simulink model "servomotor_pendul"  (Simulink 6.6)
settings: Solver=ode45  StartTime=0.0  StopTime=10  RelTol=1e-3
settings Model: Creator=123  LastModifiedBy=123

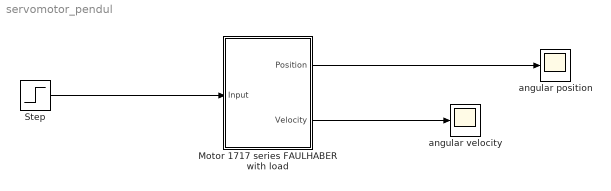
== system servomotor_pendul ==
  Motor 1717 series FAULHABER with load : Subsystem
  Step : Step  SampleTime=0
  angular position : Scope
  angular velocity : Scope
      settings: SaveName=ScopeData2
  wires:
  Step/1 -> Motor 1717 series FAULHABER with load/1(Input)
  Motor 1717 series FAULHABER with load/1(Position) -> angular position/1
  Motor 1717 series FAULHABER with load/2(Velocity) -> angular velocity/1

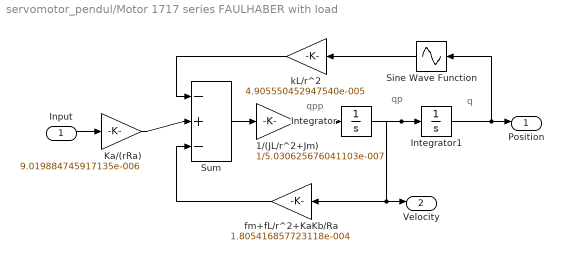
== system servomotor_pendul/Motor 1717 series FAULHABER with load ==
  note: qpp
  note: qp
  note: q
  Input : Inport
  1/(JL/r^2+Jm) : Gain  Gain=1/5.030625676041103e-007
  Integrator : Integrator
  Integrator1 : Integrator
  Ka/(rRa) : Gain  Gain=9.019884745917135e-006
  Sine Wave Function : Sin  Orientation=left  TimeSource=Use external signal  SampleTime=0
  Sum : Sum  Inputs=|-+-
  fm+fL/r^2+KaKb/Ra : Gain  Orientation=left  Gain=1.805416857723118e-004
  kL/r^2 : Gain  Orientation=left  Gain=4.905550452947540e-005
  Position : Outport
  Velocity : Outport  Port=2
  wires:
  Sum/1 -> 1/(JL/r^2+Jm)/1
  Integrator/1 -> Integrator1/1, fm+fL/r^2+KaKb/Ra/1, Velocity/1
  1/(JL/r^2+Jm)/1 -> Integrator/1
  Integrator1/1 -> Sine Wave Function/1, Position/1
  Sine Wave Function/1 -> kL/r^2/1
  fm+fL/r^2+KaKb/Ra/1 -> Sum/3
  Ka/(rRa)/1 -> Sum/2
  kL/r^2/1 -> Sum/1
  Input/1 -> Ka/(rRa)/1
